simulink model "MPPT"  (R2024b)
settings: Solver=VariableStepAuto  StartTime=0.0  StopTime=10.0  FixedStep=1e-6  RelTol=1e-4
libraries: spsSeriesRLCBranchLib x4, spsCurrentMeasurementLib x1, spsDiodeLib x1, spsMosfetLib x1, spsPVArrayLib x1, simulink x1, spsVoltageMeasurementLib x1, spspowerguiLib x1
settings Model: Creator=VICTUS  LastModifiedBy=VICTUS
settings SolverCC: ZeroCrossAlgorithm=Adaptive
settings DebuggingCC: IgnoredZcDiagnostic=none

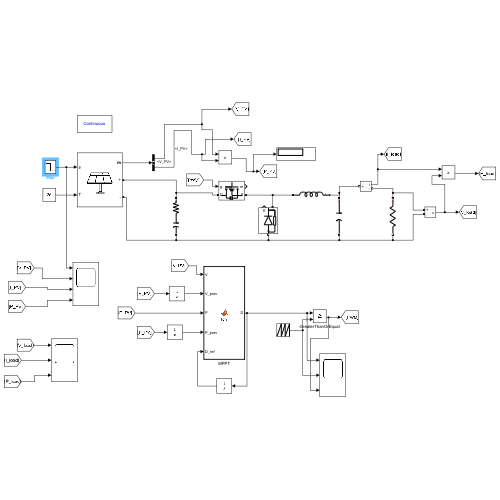
[thumbnail: Simulink's stored preview of the top-level diagram]
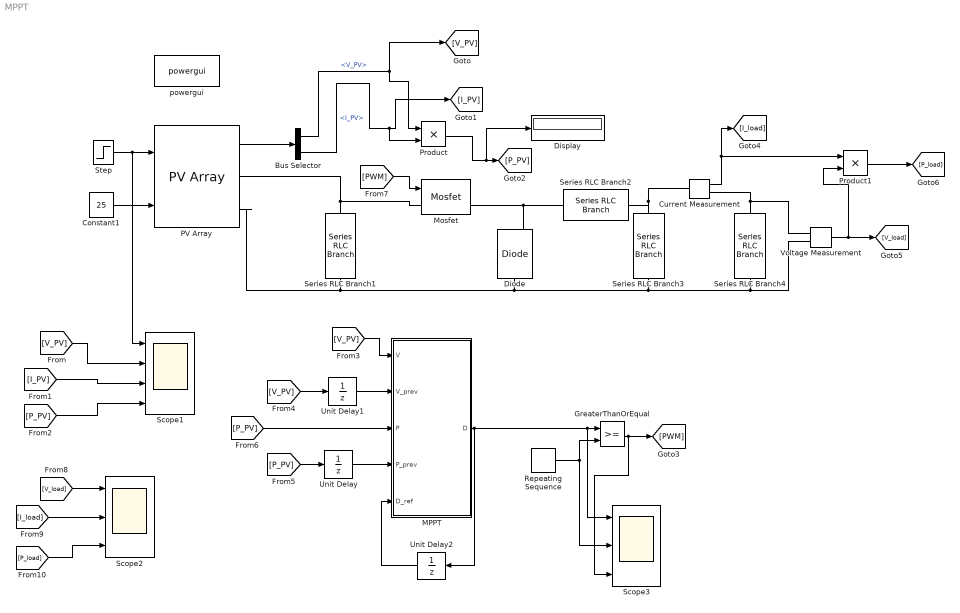
== system MPPT ==
  Bus Selector : BusSelector  OutputSignals=V_PV,I_PV
  Constant1 : Constant  Value=25
  Current Measurement : spsCurrentMeasurementLib/Current Measurement  PhasorSimulation=off  OutputType=Complex  PSBequivalent=0
  Diode : spsDiodeLib/Diode  Ron=0.001  Lon=0  Vf=0.8  IC=0  UseSnubber=0  Rs=500  Cs=250e-9  Measurements=on
  Display : Display
  GreaterThanOrEqual : RelationalOperator  OutDataTypeStr=boolean  ZeroCross=off  RndMeth=Simplest  InputSameDT=off
  MPPT : MATLAB Function  TreatAsAtomicUnit=on
  Mosfet : spsMosfetLib/Mosfet  Ron=0.1  Lon=0  Rd=0.01  Vfd=0  IC=0  Rs=1e5  Cs=inf  Measurements=on
  PV Array : spsPVArrayLib/PV Array  Npar=1  Nser=2  PlotType=array @ 1000 W/m2 & specified temperatures  S_vec="[ 1000  500  100 ]"  Temp_C_vec="[ 45 25  ]"  ModuleName=User-defined  PlotWhenSelected=off  Pm=213.15  Ncell=60  Voc=36.3  Isc=7.84  Vm=29  Im=7.35  beta_Voc_pc=-0.36099  alpha_Isc_pc=0.102  beta_Voc=-0.13104  alpha_Isc=0.0079968  IL=7.8654  I0=2.9273e-10  nI=0.98119  Rsh=313.0553  Rs=0.39381  RobustModel=off  RobustCellTemperature=313.3991  BAL=on  Tc=1e-6  Tfilter=5e-5
  Product : Product
  Product1 : Product
  Repeating Sequence : simulink/Sources/Repeating Sequence  rep_seq_t=[0 1e-3]  rep_seq_y=[0 1]
  Scope1 : Scope  NumInputPorts=4
  Scope2 : Scope  NumInputPorts=3
  Scope3 : Scope  NumInputPorts=3
  Series RLC Branch1 : spsSeriesRLCBranchLib/Series RLC Branch  LConnTagsString=__new0  RConnTagsString=__new0  BranchType=RC  Resistance=0.001  Inductance=1e-3  SetiL0=off  InitialCurrent=0  Capacitance=1000e-6  Setx0=off  InitialVoltage=0  Measurements=None
  Series RLC Branch2 : spsSeriesRLCBranchLib/Series RLC Branch  LConnTagsString=__new0  RConnTagsString=__new0  BranchType=L  Resistance=0.001  Inductance=10e-3  SetiL0=off  InitialCurrent=0  Capacitance=1000e-6  Setx0=off  InitialVoltage=0  Measurements=None
  Series RLC Branch3 : spsSeriesRLCBranchLib/Series RLC Branch  LConnTagsString=__new0  RConnTagsString=__new0  BranchType=C  Resistance=0.001  Inductance=1e-3  SetiL0=off  InitialCurrent=0  Capacitance=300e-6  Setx0=off  InitialVoltage=0  Measurements=None
  Series RLC Branch4 : spsSeriesRLCBranchLib/Series RLC Branch  LConnTagsString=__new0  RConnTagsString=__new0  BranchType=R  Resistance=1  Inductance=1e-3  SetiL0=off  InitialCurrent=0  Capacitance=1000e-6  Setx0=off  InitialVoltage=0  Measurements=None
  Step : Step  Time=5  Before=1000  After=400  SampleTime=0
  Unit Delay : UnitDelay  SampleTime=-1  HasFrameUpgradeWarning=on
  Unit Delay1 : UnitDelay  SampleTime=-1  HasFrameUpgradeWarning=on
  Unit Delay2 : UnitDelay  InitialCondition=0.5  SampleTime=-1  HasFrameUpgradeWarning=on
  Voltage Measurement : spsVoltageMeasurementLib/Voltage Measurement  PhasorSimulation=off  OutputType=Complex  PSBequivalent=0
  powergui : spspowerguiLib/powergui  Priority=1  SimulationMode=Continuous  SampleTime=50e-6  frequency=60  Iterations=50  frequencyindice=0  Pbase=100e6  ErrMax=1e-4  UnitsV=kV  UnitsW=MW  buscounter=0  FunctionMessages=off  echomessages=off  EnableUseOfTLC=off  CurrentSourceSwitches=off  DisableSnubberDevices=off  DisableRonSwitches=off  DisableVfSwitches=off  DisplayEquations=off  AutomaticDiscreteSolvers=off  SolverType=Tustin/Backward Euler (TBE)  Interpol=off  ExternalGateDelay=off  methode=off  Ts=100  x0status=blocks  SPID=on  SwTol=0  HookPort=off  NonlinearTolerance=1e-4  nMaxIteration=100  ContinueOnMaxIteration=off  RestoreLinks=warning  ResistiveCurrentMeasurement=off  Frange=[0:2:500]  Ylog=off  Xlog=on  ShowGrid=off  save=off  variable=ZData  structure=0  ZoomFFT=off  StartTime=0.0  cycles=1  DisplayStyle=1  fundamental=60  FreqAxis=off  MaxFrequency=1000  frequencyindicesteady=1  RmsSteady=1  display=off
  wires:
  Step/1 -> Scope1/1, PV Array/1
  Constant1/1 -> PV Array/2
  PV Array/1 -> Bus Selector/1
  Bus Selector/1 -> [V_PV], Product/1  "<V_PV>"
  Bus Selector/2 -> [I_PV], Product/2  "<I_PV>"
  Product/1 -> Display/1, [P_PV]
  [V_PV] -> Scope1/2
  [I_PV] -> Scope1/3
  [P_PV] -> Scope1/4
  Unit Delay/1 -> MPPT/4(P_prev)
  Unit Delay1/1 -> MPPT/2(V_prev)
  [V_PV] -> MPPT/1(V)
  [V_PV] -> Unit Delay1/1
  [P_PV] -> Unit Delay/1
  [P_PV] -> MPPT/3(P)
  MPPT/1(D) -> Unit Delay2/1, Scope3/1, GreaterThanOrEqual/1
  Repeating Sequence/1 -> Scope3/2, GreaterThanOrEqual/2
  GreaterThanOrEqual/1 -> Scope3/3, [PWM]
  Current Measurement/1 -> [I_load], Product1/1
  Voltage Measurement/1 -> Product1/2, [V_load]
  Product1/1 -> [P_load]
  [V_load] -> Scope2/1
  [I_load] -> Scope2/2
  [P_load] -> Scope2/3
  [PWM] -> Mosfet/1
  Unit Delay2/1 -> MPPT/5(D_ref)
  connections:
  Series RLC Branch1/LConn1 -- PV Array/RConn1 -- Mosfet/LConn1
  Mosfet/RConn1 -- Series RLC Branch2/RConn1 -- Diode/RConn1
  Series RLC Branch3/LConn1 -- Series RLC Branch2/LConn1 -- Current Measurement/LConn1
  PV Array/RConn2 -- Diode/LConn1 -- Voltage Measurement/LConn2 -- Series RLC Branch4/RConn1 -- Series RLC Branch3/RConn1 -- Series RLC Branch1/RConn1
  Current Measurement/RConn1 -- Voltage Measurement/LConn1 -- Series RLC Branch4/LConn1

== matlab function MPPT/MPPT ==
  data: V input; D output; V_prev input; P input; P_prev input; D_ref input
function D = fcn(V, V_prev, P, P_prev, D_ref)

    step = 0.01; 

    if (P > P_prev)
        % Power increased: Keep moving in same direction
        if (V > V_prev)
            % Voltage is rising. To keep it rising in a BUCK, DECREASE D.
            D = D_ref - step; 
        else
            % Voltage is dropping. To keep it dropping in a BUCK, INCREASE D.
            D = D_ref + step;
        end
    else
        % Power decreased: Reverse direction
        if (V > V_prev)
            % Voltage rose but power dropped. We are to the right of peak. Need to LOWER V.
            % In BUCK, to lower V, INCREASE D.
            D = D_ref + step;
        else
            % Voltage fell and power dropped. We are to the left of peak. Need to RAISE V.
            % In BUCK, to raise V, DECREASE D.
            D = D_ref - step;
        end
    end
    
    % Saturation limits
    if D > 0.9
        D = 0.9;
    elseif D < 0.1
        D = 0.1;
    end
end
